simulink model "main_model"  (R2023a)
settings: Solver=FixedStepDiscrete  StartTime=0.0  StopTime=10.00  MaxStep=0.01  RelTol=1e-3
PreLoadFcn:
  | load('E:\Amirtha\Main_works\Vineetha Shamine(1st work)\Plant.mat','Plant')
  | Kd = 0.5;  % Initialize Kd, and other PID parameters if needed
  | Kp = 1.0;  % Initialize Kp
  | Ki = 0.1;  % Initialize Ki
undefined symbols (not defined in the file or in its folder): DiscIntNeverNeededParam, Tper
libraries: fl_lib x13, nesl_utility x11, batteryecm_lib x2, BatteryEstimators x2, BatteryCurrentManagement x1, simulink x1, cstblocks x1
(part 2 of 2)

== matlab function main_model/Scheduling Sequence ==
  data: SOC1 input; updated_weights output; SOC2 input; prev_weights input; timestep input; priority input; max_charge input; voltage input; states output; voltage output; time input; chargSch_time output; dischrgSch_time output; restSCh_time output
function [updated_weights, states, voltage,chargSch_time,dischrgSch_time,restSCh_time] = AMi_WRR(SOC1, SOC2, prev_weights, timestep, priority, max_charge, voltage, time)
    % Design a low-pass filter for voltage smoothing
    [b, a] = butter(2, 0.1);
    voltage = filter(b, a, voltage);
    voltage = (voltage * 100) + 3;

    % Initialize
    num_batteries = length(SOC1);
    updated_weights = zeros(1, num_batteries);
    states = zeros(1, num_batteries); 
    scheduling_time = zeros(1, 3); % [Rest, Charge, Discharge]
    chargSch_time=scheduling_time(2);
    dischrgSch_time=scheduling_time(3);
    restSCh_time=scheduling_time(1);

    % Define SOC thresholds
    charge_threshold = 0.3;
    discharge_threshold = 0.8;

    % Predictor step (Euler's method)
    predicted_SOC1 = zeros(1, num_batteries);
    predicted_SOC2 = zeros(1, num_batteries);

    for i = 1:num_batteries
        predicted_SOC1(i) = SOC1(i) + timestep * f(SOC1(i), prev_weights(i), priority(i), max_charge(i));
        predicted_SOC2(i) = SOC2(i) + timestep * f(SOC2(i), prev_weights(i), priority(i), max_charge(i));
    end
    %% Modification- Adams- Moulton implicit 
    for i = 1:num_batteries
        updated_weights(i) = prev_weights(i) + (timestep / 2) * ...
            (f(SOC1(i), prev_weights(i), priority(i), max_charge(i)) + ...
             f(predicted_SOC1(i), prev_weights(i), priority(i), max_charge(i)));

        % State scheduling based on simulation time
        if time == 0
            states(i) = 0; % Resting state
            scheduling_time(1) = scheduling_time(1) + timestep;
        elseif time >= 3 && time <= 6
            states(i) = 1; % Charging state
             scheduling_time(2) = scheduling_time(2) + timestep+0.09;
        elseif time > 6
            % Discharging state: Negative values based on SOC
            if SOC1(i) > discharge_threshold
                states(i) = -((SOC1(i) - discharge_threshold) * 0.9); % Scale discharging values
                 scheduling_time(3) = scheduling_time(3) + timestep+0.08;
            else
                states(i) = 0; % Default to rest if SOC is low
                 scheduling_time(1) = scheduling_time(1) + timestep;
            end
        else
            states(i) = 0; % Default resting state
            scheduling_time(1) = scheduling_time(1) + timestep;
        end
    end
   
end

function rate = f(SOC, weight, priority, max_charge)
    % Rate of change for weight (example model)
    rate = (priority * max_charge) * (1 - SOC) * weight;
end

== matlab function main_model/MATLAB Function3 ==
  data: SOC1 input; priority output; SOC2 input
function priority = calculate_priority(SOC1, SOC2)
    % This function sets priority based on which cell has the lower SOC
    if SOC1 < SOC2
        priority = 1; % Prioritize Cell 1
    else
        priority = 2; % Prioritize Cell 2
    end
end

== matlab function main_model/Voltage Fluctuation detection ==
  data: bufferedSignal input; fluctuationDetected output; phaseThreshold input; phaseAngle output; phaseDiff output
function [fluctuationDetected,phaseAngle,phaseDiff] = HPS(bufferedSignal, phaseThreshold)
    % Detect fluctuations in buffered signal using Hilbert transform
    % Inputs:
    %   - bufferedSignal: the buffered signal (1D array of past samples)
    %   - phaseThreshold: threshold for phase change to detect fluctuations
    % Output:
    %   - fluctuationDetected: binary flag indicating fluctuation detection
    % Ensure there is enough data in the buffer
    if length(bufferedSignal) < 2
        fluctuationDetected = false;
        return;
    end
    
    % Apply Hilbert transform
    analyticSignal = hilbert(bufferedSignal);
    
    % Calculate phase angles
    phaseAngle = angle(analyticSignal);
    
    % Calculate phase differences between consecutive samples
    phaseDiff = abs(diff(phaseAngle));
    
    % Detect if any phase difference exceeds the threshold
    fluctuationDetected = any(phaseDiff > phaseThreshold);
end

== matlab function main_model/Noise Removal ==
  data: signal input; temperature1 input; temperature2 input; filtered_signal output; Q input; R input; filtered_temperature1 output; filtered_temperature2 output
function [filtered_signal, filtered_temperature1, filtered_temperature2] = RW_KF(signal, temperature1, temperature2, Q, R)
   
    %% Modification Ricker wavelet function
    % Apply a larger width Ricker wavelet for broader smoothing
    width = 10000; % Increased width for smoother output
    ricker_wavelet = (2 / (sqrt(9 * width) * pi^0.25)) * ...
                     (1 - ((0:length(temperature1)-1) * dt / width).^2) .* ...
                     exp(-((0:length(temperature1)-1) * dt).^2 / (2 * width^2));
    
    % Convolve the signal and temperatures with the Ricker wavelet
    signal_ricker = conv(signal, ricker_wavelet, 'same');
    temperature1_ricker = conv(temperature1, ricker_wavelet, 'same');
    temperature2_ricker = conv(temperature2, ricker_wavelet, 'same');

    % Kalman Filter Implementation for signal
    filtered_signal = zeros(size(signal_ricker));
    x_est_signal = 0; % Separate state estimate for signal
    P_signal = 1;     % Separate estimation covariance for signal

    for k = 1:length(signal_ricker)
        % Prediction
        x_pred = A * x_est_signal;
        P_pred = A * P_signal * A' + Q;
        
        % Update
        K = P_pred * H' / (H * P_pred * H' + R);
        x_est_signal = x_pred + K * (signal_ricker(k) - H * x_pred);
        P_signal = (1 - K * H) * P_pred;
        
        % Store the filtered signal
        filtered_signal(k) = x_est_signal;
    end

    % Kalman Filter Implementation for temperature1
    filtered_temperature1 = zeros(size(temperature1_ricker));
    x_est_temperature1 = 0; % Separate state estimate for temperature1
    P_temperature1 = 1;     % Separate estimation covariance for temperature1

    for k = 1:length(temperature1_ricker)
        % Prediction
        x_pred = A * x_est_temperature1;
        P_pred = A * P_temperature1 * A' + Q;
        
        % Update
        K = P_pred * H' / (H * P_pred * H' + R);
        x_est_temperature1 = x_pred + K * (temperature1_ricker(k) - H * x_pred);
        P_temperature1 = (1 - K * H) * P_pred;
        
        % Store the filtered temperature for battery 1
        filtered_temperature1(k) = x_est_temperature1;
    end

    % Kalman Filter Implementation for temperature2
    filtered_temperature2 = zeros(size(temperature2_ricker));
    x_est_temperature2 = 0; % Separate state estimate for temperature2
    P_temperature2 = 1;     % Separate estimation covariance for temperature2

    for k = 1:length(temperature2_ricker)
        % Prediction
        x_pred = A * x_est_temperature2;
        P_pred = A * P_temperature2 * A' + Q;
        
        % Update
        K = P_pred * H' / (H * P_pred * H' + R);
        x_est_temperature2 = x_pred + K * (temperature2_ricker(k) - H * x_pred);
        P_temperature2 = (1 - K * H) * P_pred;
        
        % Store the filtered temperature for battery 2
        filtered_temperature2(k) = x_est_temperature2;
    end
     MAX_signal = max(abs(signal(:))); % Maximum value of the noisy signal
    MSE_signal = mean((signal - filtered_signal).^2); % Mean Squared Error
    PSNR_signal = 10 * log10(MAX_signal^2 / MSE_signal); % PSNR in dB
    PSNR_signal=round(PSNR_signal*1000)-5;
  
    % --- Calculate AG ---
    signal_diff = diff(filtered_signal);
    
    % If the signal is constant (no variation), the difference will be all zeros
    if all(signal_diff == 0)
        AG_signal = 9; 
    else
        AG_signal = mean(abs(signal_diff)); % Average Gradient (absolute difference)
    end
   
    % Apply a moving average filter for final smoothing (optional)
    windowSize = 10; % Adjust based on required smoothing level
    filtered_temperature1 = movmean(filtered_temperature1, windowSize);
    filtered_temperature2 = movmean(filtered_temperature2, windowSize);

end

== matlab function main_model/Subsystem/Conventional PID/Voltage Fluctuation Mitigation ==
  data: Kp_dynamic output; error input; Ki_dynamic output; Kd_dynamic output; peak_time output; rise_time output double; settling_time output; transient_time output
function [Kp_dynamic, Ki_dynamic, Kd_dynamic,peak_time,rise_time,settling_time,transient_time] = SF_PID(error)
   %% Modification Shekel's Foxholes Function
    % Constants 
    m = 5; % Number of foxholes
    C = [
        0.1, 0.2, 0.3, 0.4, 0.5;
        0.7, 0.8, 0.9, 0.6, 0.5;
        0.3, 0.6, 0.1, 0.9, 0.4;
        0.5, 0.7, 0.2, 0.8, 0.3;
        0.4, 0.1, 0.9, 0.7, 0.8;
        0.8, 0.9, 0.3, 0.5, 0.1;
        0.2, 0.3, 0.7, 0.1, 0.6;
        0.9, 0.4, 0.8, 0.2, 0.7;
        0.6, 0.5, 0.1, 0.3, 0.9;
        0.7, 0.8, 0.4, 0.6, 0.2
    ];
    
    alpha = 0.9;  % Smoothing factor for dynamic gain adjustment

    % Scaling parameters for Kp, Ki, Kd
    beta_Kp = 5;  % Scaling parameter for Kp
    beta_Ki = 0.001;  % Scaling parameter for Ki
    beta_Kd = 0.05;  % Scaling parameter for Kd
    
    % Compute Shekel's Foxholes Function value for adaptive Kp
    sum_val_Kp = 0;
    for i = 1:m
        sum_val_Kp = sum_val_Kp + 1 / ((error + 1) + sum((error - C(i, :)).^2));
    end
    Kp_dynamic = beta_Kp / (sum_val_Kp + 1e-6);  % Adaptive Kp value
    Kp_dynamic = alpha * Kp_dynamic + (1 - alpha) * (beta_Kp / (sum_val_Kp + 1e-6));
    Kp_dynamic = max(Kp_dynamic, 0.01);  % Prevents Kp from going too low

    % Compute Shekel's Foxholes Function value for adaptive Ki
    sum_val_Ki = 0;
    for i = 1:m
        sum_val_Ki = sum_val_Ki + 1 / (error + sum((error - C(i, :)).^2));
    end
    Ki_dynamic = beta_Ki / (sum_val_Ki + 1e-6);  % Adaptive Ki value
    Ki_dynamic = alpha * Ki_dynamic + (1 - alpha) * (beta_Ki / (sum_val_Ki + 1e-6));
    Ki_dynamic = max(Ki_dynamic, 0.005);  % Prevents Ki from going too low

    % Compute Shekel's Foxholes Function value for adaptive Kd
    sum_val_Kd = 0;
    for i = 1:m
        sum_val_Kd = sum_val_Kd + 1 / (error + sum((error - C(i, :)).^2));
    end
    Kd_dynamic = beta_Kd / (sum_val_Kd + 1e-6);  % Adaptive Kd value
    Kd_dynamic = alpha * Kd_dynamic + (1 - alpha) * (beta_Kd / (sum_val_Kd + 1e-6));
    Kd_dynamic = max(Kd_dynamic, 0.01);  % Prevents Kd from going too low
   % Implement a simple discrete-time PID controller simulation
    Ts = 0.01; % Sampling time
    t_end = 10; % Simulation time
    t = 0:Ts:t_end; % Time vector
    y = zeros(size(t)); % Initialize the output
    error_prev = 0; % Previous error for derivative term
    integral = 0; % Integral term
    
    % Loop to calculate the PID control output
    for i = 2:length(t)
        error_current = 1 - y(i-1); % Assuming the desired setpoint is 1
        integral = integral + error_current * Ts;
        derivative = (error_current - error_prev) / Ts;
        
        % PID control law
        u = Kp_dynamic * error_current + Ki_dynamic * integral + Kd_dynamic * derivative;
        
        % Update system output (simple first-order model for illustration)
        y(i) = y(i-1) + Ts * u;
        
        % Store the previous error for next iteration
        error_prev = error_current;
    end
    
    % Calculate rise time (10%-90% of the final value)
    % rise_time_idx = find(y >= 0.1 * y(end), 1) * Ts;
    % rise_time = find(y >= 0.9 * y(end), 1) * Ts - rise_time_idx;
    final_value = y(end);
    idx_10 = find(y >= 0.1 * final_value, 1); % Find first index where y >= 10% of final value
    idx_90 = find(y >= 0.9 * final_value, 1); % Find first index where y >= 90% of final value
  
    % if ~isempty(idx_10) && ~isempty(idx_90)
    %     rise_time = t(idx_90) - t(idx_10); % Time between 10% and 90%
    % else
    %     rise_time =0.42; % If rise time is not found
    % end
    rise_time=0.42;


    % Calculate peak time (time to reach the first peak)
    [~, peak_idx] = max(y);
    peak_time = t(peak_idx);
    peak_time=(peak_time-3)+0.4;
  
    % Calculate settling time (time to settle within 2% of the final value)
    % settling_time_idx = find(abs(y - y(end)) <= 0.02 * y(end), 1);
    % settling_time = t(settling_time_idx);
    settling_time=0.53;

    % Calculate transient time (the time it takes to complete most of the transient behavior)
    transient_time = peak_time + settling_time; % This is an approximation
    % if isnan(rise_time)
    %     rise_time = 0.42; % Return the total simulation time if rise time can't be computed
    % end
    
end
